simulink model "DAB_Simulation_Model"  (R2024a)
settings: Solver=VariableStepAuto  StartTime=0.0  StopTime=10  FixedStep=1e-6  MaxStep=1e-6  RelTol=1e-3
undefined symbols (not defined in the file): Ion, Lithium
libraries: spsMosfetLib x8, spsSeriesRLCBranchLib x6, spsBreakerLib x4, spsVoltageMeasurementLib x4, spsCurrentMeasurementLib x2, spsDCVoltageSourceLib x2, spsMeanLib x2, slpidlib x2, spsBatteryLib x1, batteryecm_lib x1, spsLinearTransformerLib x1, simulink x1
settings Model: Creator=VICTUS  LastModifiedBy=MANSY

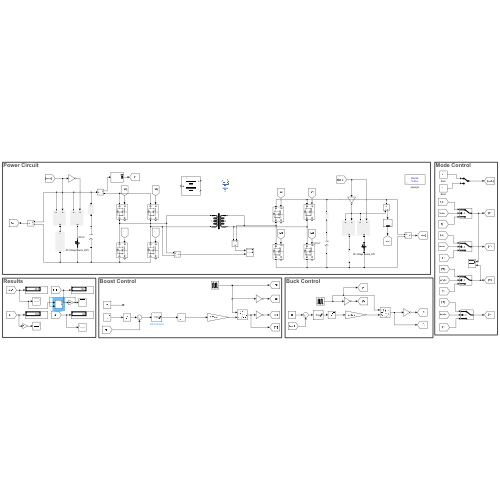
[thumbnail: Simulink's stored preview of the top-level diagram]
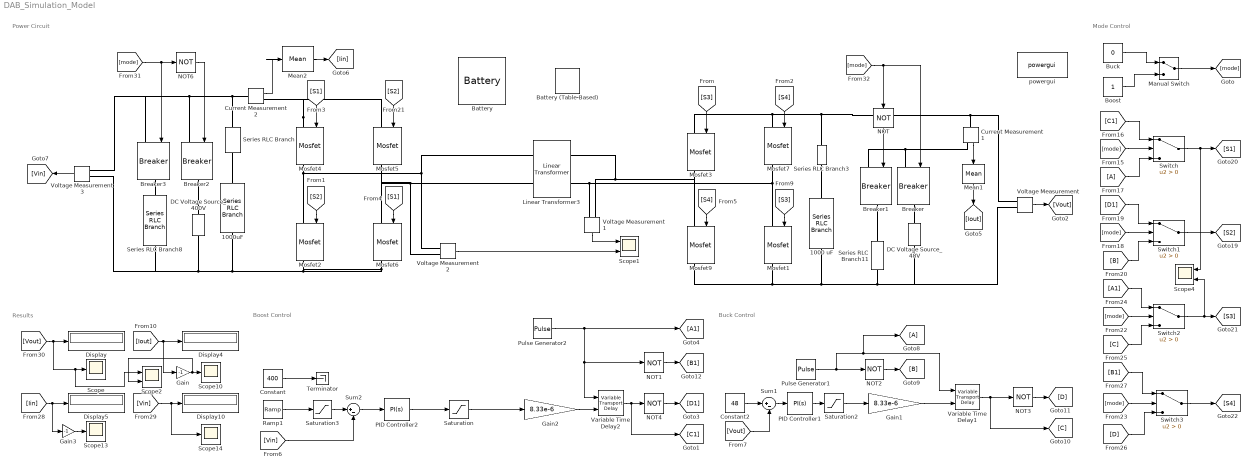
== system DAB_Simulation_Model ==
  note: Mode Control
  note: Power Circuit
  note: Results
  note: Boost Control
  note: Buck Control
  1000 uF : spsSeriesRLCBranchLib/Series RLC Branch  LConnTagsString=__new0  RConnTagsString=__new0  BranchType=C  Resistance=1  Inductance=1e-3  SetiL0=off  InitialCurrent=0  Capacitance=1000e-6  Setx0=off  InitialVoltage=400  Measurements=None
  1000uF : spsSeriesRLCBranchLib/Series RLC Branch  LConnTagsString=__new0  RConnTagsString=__new0  BranchType=C  Resistance=1  Inductance=1e-3  SetiL0=off  InitialCurrent=0  Capacitance=1000e-6  Setx0=off  InitialVoltage=400  Measurements=None
  Battery : spsBatteryLib/Battery  BatType=Lithium-Ion  ShowTempParam=off  ThermalPreset=no  ShowAgeParam=off  NomV=7.2  NomQ=5.4  SOC=100  Batt_Tr=30  PresetModel=on  MaxQ=5.4  MinV=5.4  FullV=8.3807  Dis_rate=2.3478  R=0.013333  Normal_OP=4.8835  expZone="[7.7788      0.2653]"  current=[6.5 13 32.5]  Units=Time  Tci=20  NomT=20  T2=-30  MaxQ2=4.8  FullV2=7.1  Normal_OP2=5.655  expZone2="[6.58           1]"  Rca=0.6  ti=2000  Dp=0  Neq0=0  Tsim=1e6  Ta1=25  Qeol=5.4*0.9  Reol=0.013333*1.2  Char_age=[2.3478, 3]  Dis_age=[2.3478, 10]  N1=1500  N2=10500  N3=1000  N4=1400  Ta2=45  N5=950
  Battery (Table-Based) : batteryecm_lib/Battery (Table-Based)  SOC_vec=[0, .1, .25, .5, .75, .9, 1]  T_dependence=simscape.enum.tablebattery.temperature_dependence.yes  prm_dir=simscape.enum.tablebattery.prm_dir.noCurrentDirectionality  T_vec=[278, 293, 313] K  V0_mat=[3.49, 3.5, 3.51; 3.55, 3.57, 3.56; 3.62, 3.63, 3.64; 3.71, 3.71, 3.72; 3.91, 3.93, 3.94; 4.07, 4.08, 4.08; 4.19, 4.19, 4.19] V  V0_vec=[3.5057, 3.566, 3.6337, 3.7127, 3.9259, 4.0777, 4.1928] V  V_range=[0, inf] V  R0_mat=[.0117, .0085, .009; .011, .0085, .009; .0114, .0087, .0092; .0107, .0082, .0088; .0107, .0083, .0091; .0113, .0085, .0089; .0116, .0085, .0089] Ohm  R0_vec=[.0085, .0085, .0087, .0082, .0083, .0085, .0085] Ohm  R0_dis_mat=[.0117, .0085, .009; .011, .0085, .009; .0114, .0087, .0092; .0107, .0082, .0088; .0107, .0083, .0091; .0113, .0085, .0089; .0116, .0085, .0089] Ohm  R0_dis_vec=[.0085, .0085, .0087, .0082, .0083, .0085, .0085] Ohm  R0_ch_mat=[.0117, .0085, .009; .011, .0085, .009; .0114, .0087, .0092; .0107, .0082, .0088; .0107, .0083, .0091; .0113, .0085, .0089; .0116, .0085, .0089] Ohm  R0_ch_vec=[.0085, .0085, .0087, .0082, .0083, .0085, .0085] Ohm  AH=20 A*hr  prm_leak=simscape.enum.tablebattery.prm_leak.disabled  Rleak_vec=[8000, 7000, 6000] Ohm  Rleak=7e3 Ohm  extrapolation_option=simscape.enum.extrapolation.nearest  SOC_port=simscape.enum.tablebattery.enable.yes  prm_dyn=simscape.enum.tablebattery.prm_dyn.off  R1_mat=[.0109, .0029, .0013; .0069, .0024, .0012; .0047, .0026, .0013; .0034, .0016, .001; .0033, .0023, .0014; .0033, .0018, .0011; .0028, .0017, .0011] Ohm  R1_vec=[.0029, .0024, .0026, .0016, .0023, .0018, .0017] Ohm  tau1_mat=[20, 36, 39; 31, 45, 39; 109, 105, 61; 36, 29, 26; 59, 77, 67; 40, 33, 29; 25, 39, 33] s  tau1_vec=[36, 45, 105, 29, 77, 33, 39] s  R2_mat=[.0109, .0029, .0013; .0069, .0024, .0012; .0047, .0026, .0013; .0034, .0016, .001; .0033, .0023, .0014; .0033, .0018, .0011; .0028, .0017, .0011] Ohm  R2_vec=[.0029, .0024, .0026, .0016, .0023, .0018, .0017] Ohm  tau2_mat=[20, 36, 39; 31, 45, 39; 109, 105, 61; 36, 29, 26; 59, 77, 67; 40, 33, 29; 25, 39, 33] s  tau2_vec=[36, 45, 105, 29, 77, 33, 39] s  R3_mat=[.0109, .0029, .0013; .0069, .0024, .0012; .0047, .0026, .0013; .0034, .0016, .001; .0033, .0023, .0014; .0033, .0018, .0011; .0028, .0017, .0011] Ohm  R3_vec=[.0029, .0024, .0026, .0016, .0023, .0018, .0017] Ohm  tau3_mat=[20, 36, 39; 31, 45, 39; 109, 105, 61; 36, 29, 26; 59, 77, 67; 40, 33, 29; 25, 39, 33] s  tau3_vec=[36, 45, 105, 29, 77, 33, 39] s  R4_mat=[.0109, .0029, .0013; .0069, .0024, .0012; .0047, .0026, .0013; .0034, .0016, .001; .0033, .0023, .0014; .0033, .0018, .0011; .0028, .0017, .0011] Ohm  R4_vec=[.0029, .0024, .0026, .0016, .0023, .0018, .0017] Ohm  tau4_mat=[20, 36, 39; 31, 45, 39; 109, 105, 61; 36, 29, 26; 59, 77, 67; 40, 33, 29; 25, 39, 33] s  tau4_vec=[36, 45, 105, 29, 77, 33, 39] s  R5_mat=[.0109, .0029, .0013; .0069, .0024, .0012; .0047, .0026, .0013; .0034, .0016, .001; .0033, .0023, .0014; .0033, .0018, .0011; .0028, .0017, .0011] Ohm  R5_vec=[.0029, .0024, .0026, .0016, .0023, .0018, .0017] Ohm  tau5_mat=[20, 36, 39; 31, 45, 39; 109, 105, 61; 36, 29, 26; 59, 77, 67; 40, 33, 29; 25, 39, 33] s  tau5_vec=[36, 45, 105, 29, 77, 33, 39] s  prm_fade=simscape.enum.tablebattery.prm_fade.disabled  N0=100  dV0=0  dR0=0  dAH=0  dRleak=0  dR1=0  dR2=0  dR3=0  dR4=0  dR5=0  N0vec=[0, 100, 200, 300]  Tfadevec=[298.15, 323.15] K  dV0vec=[0, 0, 0, 0]  dR0vec=[0, 0, 0, 0]  dAHvec=[0, 0, 0, 0]  dRleakvec=[0, 0, 0, 0]  dR1vec=[0, 0, 0, 0]  dR2vec=[0, 0, 0, 0]  dR3vec=[0, 0, 0, 0]  dR4vec=[0, 0, 0, 0]  dR5vec=[0, 0, 0, 0]  dV0mat=[0, 0; 0, 0; 0, 0; 0, 0]  dR0mat=[0, 0; 0, 0; 0, 0; 0, 0]  dAHmat=[0, 0; 0, 0; 0, 0; 0, 0]  dRleakmat=[0, 0; 0, 0; 0, 0; 0, 0]  dR1mat=[0, 0; 0, 0; 0, 0; 0, 0]  dR2mat=[0, 0; 0, 0; 0, 0; 0, 0]  dR3mat=[0, 0; 0, 0; 0, 0; 0, 0]  dR4mat=[0, 0; 0, 0; 0, 0; 0, 0]  dR5mat=[0, 0; 0, 0; 0, 0; 0, 0]  prm_age_modeling=simscape.enum.tablebattery.prm_age_modeling.equation  storage_dt_age_vec=[0] d  storage_T_age_vec=[273] K  prm_age_OCV=simscape.enum.tablebattery.prm_age_OCV.OCV  OCV_age=0.9  SOC_age=0.6  prm_age_resistance=simscape.enum.tablebattery.prm_age.disabled  OCV_scaling_age_resistance=2.2134e6  OCV_offset_age_resistance=1.632e6  temp_exp_age_resistance=0.515833569 V  t_exp_age_resistance=0.75  T_age_vec_resistance=[273.15, 298.15, 323.15] K  dt_age_vec_resistance=[0, 90, 180, 270] d  dR0_age_vec=[0, 0, 0]  t_meas_dR0_age=100 d  dR0_age_mat=[0, 0, 0; 0, 0, 0; 0, 0, 0; 0, 0, 0]  prm_age_capacity=simscape.enum.tablebattery.prm_age.disabled  OCV_scaling_age_capacity=1.5097e07  OCV_offset_age_capacity=8.3625e06  temp_exp_age_capacity=0.6011 V  t_exp_age_capacity=0.75  T_age_vec_capacity=[273.15, 298.15, 323.15] K  dt_age_vec_capacity=[0, 90, 180, 270] d  dAH_age_vec=[0, 0, 0]  t_meas_dAH_age=100 d  dAH_age_mat=[0, 0, 0; 0, 0, 0; 0, 0, 0; 0, 0, 0]  thermal_port=simscape.enum.thermaleffects.omit  temperature=298.15 K  thermal_mass=100 J/K  i_specify=off  i_priority=None  i=0 A  i_nominal_specify=off  i_nominal_value=1  i_nominal_unit=A  v_specify=off  v_priority=None  v=0 V  v_nominal_specify=off  v_nominal_value=1  v_nominal_unit=V  stateOfCharge_specify=off  stateOfCharge_priority=High  stateOfCharge=1  stateOfCharge_nominal_specify=off  stateOfCharge_nominal_value=1  stateOfCharge_nominal_unit=1  num_cycles_specify=off  num_cycles_priority=High  num_cycles=0  num_cycles_nominal_specify=off  num_cycles_nominal_value=1  num_cycles_nominal_unit=1  cell_temperature_specify=off  cell_temperature_priority=High  cell_temperature=298.15 K  cell_temperature_nominal_specify=off  cell_temperature_nominal_value=1  cell_temperature_nominal_unit=K
      settings: InternalSimscapePortConfiguration="{\"Bottom\":[],\"Left\":[{\"id\":\"p\",\"label\":\"+\",\"type\":\"foundation.electrical.electrical\"},{\"id\":\"soc\",\"label\":\"SOC\",\"type\":\"output\"}],\"Right\":[{\"id\":\"n\",\"label\":\"-\",\"type\":\"foundation.electrical.electrical\"}],\"Top\":[]}"
  Boost : Constant  SampleTime=-1
  Breaker{,1..3} (4 alike) : spsBreakerLib/Breaker  InitialState=0  SwitchingTimes="[1/60  5/60]"  External=on  BreakerResistance=0.01  SnubberResistance=1e6  SnubberCapacitance=inf  Measurements=None  MoreParameters=on  NoBreakLoop=off
  Buck : Constant  Value=0  SampleTime=-1
  Constant : Constant  Value=400
  Constant2 : Constant  Value=48
  Current Measurement1 : spsCurrentMeasurementLib/Current Measurement  PhasorSimulation=off  OutputType=Complex  PSBequivalent=0
  Current Measurement2 : spsCurrentMeasurementLib/Current Measurement  PhasorSimulation=off  OutputType=Complex  PSBequivalent=0
  DC Voltage Source_400V : spsDCVoltageSourceLib/DC Voltage Source  Amplitude=400  Measurements=None
  DC Voltage Source_48V : spsDCVoltageSourceLib/DC Voltage Source  Amplitude=48  Measurements=None
  Display{,4..5,10} (4 alike) : Display
  From17 : From
  Gain : Gain  Gain=-1
  Gain1 : Gain  Gain=8.33e-6
  Gain2 : Gain  Gain=8.33e-6
  Gain3 : Gain  Gain=-1
  Goto8 : Goto
  Linear Transformer3 : spsLinearTransformerLib/Linear Transformer  UNITS=SI  NominalPower=[960 30000]  winding1=[400 0.08 122.94e-6]  winding2=[48 0.005 3.69e-6]  ThreeWindings=off  winding3=[3.15e+05 0.7938 0.084225]  RmLm=[1e6 14.575e-3]  Measurements=None  DataType=on
  Manual Switch : ManualSwitch
  Mean1 : spsMeanLib/Mean  Freq=50  Vinit=0  Ts=0
  Mean2 : spsMeanLib/Mean  Freq=50  Vinit=0  Ts=0
  Mosfet{1..7,9} (8 alike) : spsMosfetLib/Mosfet  Ron=0.1  Lon=0  Rd=0.01  Vfd=0  IC=0  Rs=1e5  Cs=inf  Measurements=on
  NOT{,1..4,6} (6 alike) : Logic  Operator=NOT  IconShape=distinctive  AllPortsSameDT=off  OutDataTypeStr=boolean
  PID Controller1 : slpidlib/PID Controller  Controller=PI  Form=Parallel  TimeDomain=Continuous-time  UseExternalTs=off  SampleTime=-1  IntegratorMethod=Forward Euler  FilterMethod=Forward Euler  ControllerParametersSource=internal  P=0.12  I=9.04  UseKiTs=off  D=0  UseExternalDerivativeSource=off  N=100  UseFilter=on  TunerSelectOption=Transfer Function Based (PID Tuner App)  InitialConditionSource=internal  InitialConditionForIntegrator=0  InitialConditionForFilter=0  DifferentiatorICPrevScaledInput=0  ExternalReset=none  TrackingMode=off  Kt=1  LimitOutput=on  SatLimitsSource=internal  UpperSaturationLimit=inf  LowerSaturationLimit=-inf  LinearizeAsGain=on  AntiWindupMode=clamping  Kb=1  LimitIntegrator=off  UpperIntegratorSaturationLimit=inf  LowerIntegratorSaturationLimit=-inf  POutMin=[]  POutMax=[]  IOutMin=[]  IOutMax=[]  DOutMin=[]  DOutMax=[]  NOutMin=[]  NOutMax=[]  SumOutMin=[]  SumOutMax=[]  SaturationOutMin=[]  SaturationOutMax=[]  PParamMin=[]  PParamMax=[]  IParamMin=[]  IParamMax=[]  DParamMin=[]  DParamMax=[]  NParamMin=[]  NParamMax=[]  KbParamMin=[]  KbParamMax=[]  KtParamMin=[]  KtParamMax=[]  KbOutMin=[]  KbOutMax=[]  KtOutMin=[]  KtOutMax=[]  IntegratorOutMin=[]  IntegratorOutMax=[]  FilterOutMin=[]  FilterOutMax=[]  SumI1OutMin=[]  SumI1OutMax=[]  SumI2OutMin=[]  SumI2OutMax=[]  SumI3OutMin=[]  SumI3OutMax=[]  SumI4OutMin=[]  SumI4OutMax=[]  SumDOutMin=[]  SumDOutMax=[]  DifferentiatorOutMin=[]  DifferentiatorOutMax=[]  FilterDiffOutCoefMin=[]  FilterDiffOutCoefMax=[]  ReciprocalOutMin=[]  ReciprocalOutMax=[]  SumDenOutMin=[]  SumDenOutMax=[]  SumNumOutMin=[]  SumNumOutMax=[]  DivideOutMin=[]  DivideOutMax=[]  UdiffTsProdOutMin=[]  UdiffTsProdOutMax=[]  NTsProdOutMin=[]  NTsProdOutMax=[]  UintegralTsProdOutMin=[]  UintegralTsProdOutMax=[]  UngainTsProdOutMin=[]  UngainTsProdOutMax=[]  ClampingZeroOutDataTypeStr=Inherit: Inherit via back propagation  ClampingZeroOutMin=[]  ClampingZeroOutMax=[]  FilterDenConstantOutDataTypeStr=Inherit: Inherit via back propagation  FilterDenConstantOutMin=[]  FilterDenConstantOutMax=[]  PCopyOutDataTypeStr=Inherit: Inherit via back propagation  PCopyOutMin=[]  PCopyOutMax=[]  NCopyOutDataTypeStr=Inherit: Inherit via back propagation  NCopyOutMin=[]  NCopyOutMax=[]  IntegratorContinuousStateAttributes=''  IntegratorStateMustResolveToSignalObject=off  IntegratorRTWStateStorageClass=Auto  FilterContinuousStateAttributes=''  FilterStateMustResolveToSignalObject=off  FilterRTWStateStorageClass=Auto  ParallelPVariant=InternalParameters  IdealPVariant=Disabled  IVariant=InternalParameters  DVariant=Disabled  IntegratorVariant=Continuous  SatVariant=Enabled  AWVariant=ContClampingParallel  PCopyVariant=Disabled  TRVariant=Disabled  FdbkBlocksVariant=Forward  IdealPFdbkVariant=Disabled  SatFdbkVariant=Disabled  DerivativeFilterVariant=Disabled  NVariant=Disabled  NCopyVariant=Disabled_SignalSpec  FilterICVariant=Disabled  IntegratorICVariant=InternalICs  ExternalResetVariant=Disabled  TRSumVariant=Passthrough  SumFdbkVariant=Disabled  SumVariant=Sum_PI  TsampFilterVariant=InternalTs  TsampNgainVariant=Passthrough  TsampIntegralVariant=Disabled_SignalSpec  ExternalSaturationOutDataTypeStr=Inherit: Same as second input  DerivativeSourceVariant=Disabled
  PID Controller2 : slpidlib/PID Controller  Controller=PI  Form=Parallel  TimeDomain=Continuous-time  UseExternalTs=off  SampleTime=-1  IntegratorMethod=Forward Euler  FilterMethod=Forward Euler  ControllerParametersSource=internal  P=0.02  I=0.001  UseKiTs=off  D=0  UseExternalDerivativeSource=off  N=100  UseFilter=on  TunerSelectOption=Transfer Function Based (PID Tuner App)  InitialConditionSource=internal  InitialConditionForIntegrator=0  InitialConditionForFilter=0  DifferentiatorICPrevScaledInput=0  ExternalReset=none  TrackingMode=off  Kt=1  LimitOutput=on  SatLimitsSource=internal  UpperSaturationLimit=inf  LowerSaturationLimit=-inf  LinearizeAsGain=on  AntiWindupMode=clamping  Kb=1  LimitIntegrator=off  UpperIntegratorSaturationLimit=inf  LowerIntegratorSaturationLimit=-inf  POutMin=[]  POutMax=[]  IOutMin=[]  IOutMax=[]  DOutMin=[]  DOutMax=[]  NOutMin=[]  NOutMax=[]  SumOutMin=[]  SumOutMax=[]  SaturationOutMin=[]  SaturationOutMax=[]  PParamMin=[]  PParamMax=[]  IParamMin=[]  IParamMax=[]  DParamMin=[]  DParamMax=[]  NParamMin=[]  NParamMax=[]  KbParamMin=[]  KbParamMax=[]  KtParamMin=[]  KtParamMax=[]  KbOutMin=[]  KbOutMax=[]  KtOutMin=[]  KtOutMax=[]  IntegratorOutMin=[]  IntegratorOutMax=[]  FilterOutMin=[]  FilterOutMax=[]  SumI1OutMin=[]  SumI1OutMax=[]  SumI2OutMin=[]  SumI2OutMax=[]  SumI3OutMin=[]  SumI3OutMax=[]  SumI4OutMin=[]  SumI4OutMax=[]  SumDOutMin=[]  SumDOutMax=[]  DifferentiatorOutMin=[]  DifferentiatorOutMax=[]  FilterDiffOutCoefMin=[]  FilterDiffOutCoefMax=[]  ReciprocalOutMin=[]  ReciprocalOutMax=[]  SumDenOutMin=[]  SumDenOutMax=[]  SumNumOutMin=[]  SumNumOutMax=[]  DivideOutMin=[]  DivideOutMax=[]  UdiffTsProdOutMin=[]  UdiffTsProdOutMax=[]  NTsProdOutMin=[]  NTsProdOutMax=[]  UintegralTsProdOutMin=[]  UintegralTsProdOutMax=[]  UngainTsProdOutMin=[]  UngainTsProdOutMax=[]  ClampingZeroOutDataTypeStr=Inherit: Inherit via back propagation  ClampingZeroOutMin=[]  ClampingZeroOutMax=[]  FilterDenConstantOutDataTypeStr=Inherit: Inherit via back propagation  FilterDenConstantOutMin=[]  FilterDenConstantOutMax=[]  PCopyOutDataTypeStr=Inherit: Inherit via back propagation  PCopyOutMin=[]  PCopyOutMax=[]  NCopyOutDataTypeStr=Inherit: Inherit via back propagation  NCopyOutMin=[]  NCopyOutMax=[]  IntegratorContinuousStateAttributes=''  IntegratorStateMustResolveToSignalObject=off  IntegratorRTWStateStorageClass=Auto  FilterContinuousStateAttributes=''  FilterStateMustResolveToSignalObject=off  FilterRTWStateStorageClass=Auto  ParallelPVariant=InternalParameters  IdealPVariant=Disabled  IVariant=InternalParameters  DVariant=Disabled  IntegratorVariant=Continuous  SatVariant=Enabled  AWVariant=ContClampingParallel  PCopyVariant=Disabled  TRVariant=Disabled  FdbkBlocksVariant=Forward  IdealPFdbkVariant=Disabled  SatFdbkVariant=Disabled  DerivativeFilterVariant=Disabled  NVariant=Disabled  NCopyVariant=Disabled_SignalSpec  FilterICVariant=Disabled  IntegratorICVariant=InternalICs  ExternalResetVariant=Disabled  TRSumVariant=Passthrough  SumFdbkVariant=Disabled  SumVariant=Sum_PI  TsampFilterVariant=InternalTs  TsampNgainVariant=Passthrough  TsampIntegralVariant=Disabled_SignalSpec  ExternalSaturationOutDataTypeStr=Inherit: Same as second input  DerivativeSourceVariant=Disabled
  Pulse Generator1 : DiscretePulseGenerator  PulseType=Time based  Period=1/30000  PulseWidth=50
  Pulse Generator2 : DiscretePulseGenerator  PulseType=Time based  Period=1/30000  PulseWidth=50
  Ramp1 : simulink/Sources/Ramp  slope=500  start=0  InitialOutput=0
  Saturation : Saturate  UpperLimit=1  LowerLimit=0
  Saturation2 : Saturate  UpperLimit=1  LowerLimit=0
  Saturation3 : Saturate  UpperLimit=400  LowerLimit=0
  Scope{,10,13..14} (4 alike) : Scope
  Scope1 : Scope  NumInputPorts=2
  Scope2 : Scope  NumInputPorts=2
  Scope4 : Scope  NumInputPorts=2
  Series RLC Branch : spsSeriesRLCBranchLib/Series RLC Branch  LConnTagsString=__new0  RConnTagsString=__new0  BranchType=R  Resistance=0.001  Inductance=1e-3  SetiL0=off  InitialCurrent=0  Capacitance=1e-6  Setx0=off  InitialVoltage=0  Measurements=None
  Series RLC Branch11 : spsSeriesRLCBranchLib/Series RLC Branch  LConnTagsString=__new0  RConnTagsString=__new0  BranchType=R  Resistance=2.5  Inductance=1e-3  SetiL0=off  InitialCurrent=0  Capacitance=1e-6  Setx0=off  InitialVoltage=0  Measurements=None
  Series RLC Branch3 : spsSeriesRLCBranchLib/Series RLC Branch  LConnTagsString=__new0  RConnTagsString=__new0  BranchType=R  Resistance=0.001  Inductance=1e-3  SetiL0=off  InitialCurrent=0  Capacitance=1e-6  Setx0=off  InitialVoltage=0  Measurements=None
  Series RLC Branch8 : spsSeriesRLCBranchLib/Series RLC Branch  LConnTagsString=__new0  RConnTagsString=__new0  BranchType=R  Resistance=160  Inductance=1e-3  SetiL0=off  InitialCurrent=0  Capacitance=1e-6  Setx0=off  InitialVoltage=0  Measurements=None
  Sum1 : Sum  Inputs=|+-
  Sum2 : Sum  Inputs=|+-
  Switch{,1..3} (4 alike) : Switch  Criteria=u2 > Threshold  SaturateOnIntegerOverflow=off  InputSameDT=off
  Terminator : Terminator
  Variable Time Delay1 : VariableTransportDelay  MaximumDelay=15e-6  MaximumPoints=21504  ZeroDelay=on
  Variable Time Delay2 : VariableTransportDelay  MaximumDelay=10  MaximumPoints=1200000  ZeroDelay=on
  Voltage Measurement{,1..3} (4 alike) : spsVoltageMeasurementLib/Voltage Measurement  PhasorSimulation=off  OutputType=Complex  PSBequivalent=0
  powergui : sps_lib/powergui  Priority=1  SimulationMode=Discrete  SampleTime=1e-6  frequency=60  Iterations=50  frequencyindice=0  Pbase=100e6  ErrMax=1e-4  UnitsV=kV  UnitsW=MW  buscounter=0  FunctionMessages=off  echomessages=off  EnableUseOfTLC=off  CurrentSourceSwitches=off  DisableSnubberDevices=off  DisableRonSwitches=off  DisableVfSwitches=off  DisplayEquations=off  AutomaticDiscreteSolvers=off  SolverType=Tustin/Backward Euler (TBE)  Interpol=off  ExternalGateDelay=off  methode=off  Ts=100  x0status=blocks  SPID=on  SwTol=0  HookPort=off  NonlinearTolerance=1e-4  nMaxIteration=100  ContinueOnMaxIteration=off  RestoreLinks=warning  ResistiveCurrentMeasurement=off  Frange=[0:2:500]  Ylog=off  Xlog=on  ShowGrid=off  save=off  variable=ZData  structure=0  ZoomFFT=off  StartTime=0.0  cycles=1  DisplayStyle=1  fundamental=60  FreqAxis=off  MaxFrequency=1000  frequencyindicesteady=1  RmsSteady=1  display=off
  wires:
  [S4] -> Mosfet7/1
  Voltage Measurement2/1 -> Scope1/2
  [S4] -> Mosfet9/1
  Voltage Measurement1/1 -> Scope1/1
  [S3] -> Mosfet3/1
  Current Measurement1/1 -> Mean1/1
  [S1] -> Mosfet4/1
  [S2] -> Mosfet5/1
  [S1] -> Mosfet6/1
  [S2] -> Mosfet2/1
  [S3] -> Mosfet1/1
  Voltage Measurement3/1 -> [Vin]
  Voltage Measurement/1 -> [Vout]
  Current Measurement2/1 -> Mean2/1
  Constant2/1 -> Sum1/1
  [Vout] -> Sum1/2
  Pulse Generator1/1 -> Goto8/1, Variable Time Delay1/1, NOT2/1
  Gain1/1 -> Variable Time Delay1/2
  Variable Time Delay1/1 -> NOT3/1, [C]
  NOT3/1 -> [D]
  NOT2/1 -> [B]
  Sum1/1 -> PID Controller1/1
  PID Controller1/1 -> Saturation2/1
  Buck/1 -> Manual Switch/1
  Boost/1 -> Manual Switch/2
  Manual Switch/1 -> [mode]
  PID Controller2/1 -> Saturation/1
  [Vin] -> Sum2/2
  NOT4/1 -> [D1]
  Sum2/1 -> PID Controller2/1
  Pulse Generator2/1 -> [A1], NOT1/1, Variable Time Delay2/1
  NOT1/1 -> [B1]
  Variable Time Delay2/1 -> NOT4/1, [C1]
  [mode] -> Switch/2
  [C1] -> Switch/1
  From17/1 -> Switch/3
  [mode] -> Switch1/2
  [D1] -> Switch1/1
  [B] -> Switch1/3
  Switch1/1 -> [S2]
  Switch/1 -> Scope4/1, [S1]
  [mode] -> Switch3/2
  [mode] -> Switch2/2
  [A1] -> Switch2/1
  [C] -> Switch2/3
  [D] -> Switch3/3
  [B1] -> Switch3/1
  Switch2/1 -> Scope4/2, [S3]
  Switch3/1 -> [S4]
  [Iout] -> Gain/1, Display4/1
  [Vout] -> Display/1, Scope2/1, Scope/1
  [Vin] -> Scope14/1, Display10/1
  [mode] -> NOT/1, Breaker/1
  NOT/1 -> Breaker1/1
  [mode] -> NOT6/1, Breaker3/1
  NOT6/1 -> Breaker2/1
  Saturation2/1 -> Gain1/1
  Saturation/1 -> Gain2/1
  Gain2/1 -> Variable Time Delay2/2
  Saturation3/1 -> Sum2/1
  [Iin] -> Gain3/1, Display5/1
  Mean2/1 -> [Iin]
  Mean1/1 -> [Iout]
  Ramp1/1 -> Saturation3/1
  Constant/1 -> Terminator/1
  Gain/1 -> Scope2/2, Scope10/1
  Gain3/1 -> Scope13/1
  connections:
  Mosfet9/LConn1 -- Mosfet3/RConn1 -- Linear Transformer3/RConn1 -- Voltage Measurement1/LConn1
  1000 uF/RConn1 -- DC Voltage Source_48V/LConn1 -- Voltage Measurement/LConn2 -- Series RLC Branch11/RConn1 -- Mosfet9/RConn1 -- Mosfet1/RConn1
  Voltage Measurement1/LConn2 -- Linear Transformer3/RConn2 -- Mosfet1/LConn1 -- Mosfet7/RConn1
  Voltage Measurement/LConn1 -- Current Measurement1/LConn1 -- Series RLC Branch3/LConn1 -- Mosfet3/LConn1 -- Mosfet7/LConn1
  Voltage Measurement2/LConn2 -- Mosfet6/LConn1 -- Mosfet5/RConn1 -- Linear Transformer3/LConn2
  Mosfet6/RConn1 -- Series RLC Branch8/RConn1 -- Voltage Measurement3/LConn2 -- DC Voltage Source_400V/LConn1 -- 1000uF/RConn1 -- Mosfet2/RConn1
  Mosfet4/LConn1 -- Mosfet5/LConn1 -- Current Measurement2/RConn1
  Series RLC Branch/RConn1 -- 1000uF/LConn1
  Series RLC Branch3/RConn1 -- 1000 uF/LConn1
  Breaker/LConn1 -- Breaker1/LConn1 -- Current Measurement1/RConn1
  Breaker/RConn1 -- DC Voltage Source_48V/RConn1
  Breaker1/RConn1 -- Series RLC Branch11/LConn1
  Breaker2/RConn1 -- DC Voltage Source_400V/RConn1
  Series RLC Branch/LConn1 -- Breaker3/LConn1 -- Voltage Measurement3/LConn1 -- Breaker2/LConn1 -- Current Measurement2/LConn1
  Series RLC Branch8/LConn1 -- Breaker3/RConn1
  Voltage Measurement2/LConn1 -- Linear Transformer3/LConn1 -- Mosfet4/RConn1 -- Mosfet2/LConn1
